simulink model "pgfm_ctrl_analysis"  (R2026b)
settings: Solver=ode23t  StopTime=param.sim.simlength  FixedStep=param.sim.tc  MaxStep=param.glb_time.tc  RelTol=1e-4
values from neighbouring files (symbols this model uses):
  param = add_template_extras(param, options)    [init_model.m]
undefined symbols (not defined in the file or in its folder): magnitude
libraries: fl_lib x99, nesl_utility x59, afe_uvw_ctrl x15, discrete_time_low_pass_filter x3, threephase_inductor_lib x3, dclink_for_two_levels x3, three_phase_pwm_modulator x3, ideal_bridges_lib x3, lithium_ion_battery x1, three_phase_voltage_with_frt_emulator_mfcn x1
(part 2 of 6)

== system pgfm_ctrl_analysis/grid/power meter iec mfunc ==
  Bus Selector : BusSelector  OutputSignals=Q1p,Q1n,P1n,P1p,U1n,U1p,i_act_1n,i_react_1n,i_act_1p,i_react_1p
  Constant : Constant  Value=param.glb_time.ts_afe
  Step : Step  Time=0.025  InitialValue=1  FinalValue=0  SampleTime=0
  To Workspace1 : ToWorkspace  VariableName=i_react_1n  SampleTime=param.glb_time.ts_afe
      settings: MaxDataPoints=param.glb_time.Ns_afe
  To Workspace2 : ToWorkspace  VariableName=i_react_1p  SampleTime=param.glb_time.ts_afe
      settings: MaxDataPoints=param.glb_time.Ns_afe
  To Workspace3 : ToWorkspace  VariableName=i_act_1n  SampleTime=param.glb_time.ts_afe
      settings: MaxDataPoints=param.glb_time.Ns_afe
  To Workspace4 : ToWorkspace  VariableName=i_act_1p  SampleTime=param.glb_time.ts_afe
      settings: MaxDataPoints=param.glb_time.Ns_afe
  To Workspace5 : ToWorkspace  VariableName=u1p  SampleTime=param.glb_time.ts_afe
      settings: MaxDataPoints=param.glb_time.Ns_afe
  To Workspace6 : ToWorkspace  VariableName=u1n  SampleTime=param.glb_time.ts_afe
      settings: MaxDataPoints=param.glb_time.Ns_afe
  Zero-Order Hold{,1..5} (6 alike) : ZeroOrderHold  SampleTime=param.glb_time.ts_afe
  three_phase_power_meter_iec : MATLAB Function  TreatAsAtomicUnit=on  SystemSampleTime=param.glb_time.ts_afe
  tag scope: P1n_global=global, P1p_global=global, Q1n_global=global, Q1p_global=global
  wires:
  Bus Selector/6 -> To Workspace5/1  "<U1p>"
  Bus Selector/8 -> To Workspace1/1  "<i_react_1n>"
  Bus Selector/10 -> To Workspace2/1  "<i_react_1p>"
  Bus Selector/5 -> To Workspace6/1  "<U1n>"
  Bus Selector/4 -> [P1p_global]  "<P1p>"
  Bus Selector/2 -> [Q1n_global]  "<Q1n>"
  Bus Selector/1 -> [Q1p_global]  "<Q1p>"
  Bus Selector/7 -> To Workspace3/1  "<i_act_1n>"
  Bus Selector/9 -> To Workspace4/1  "<i_act_1p>"
  Bus Selector/3 -> [P1n_global]  "<P1n>"
  three_phase_power_meter_iec/1(m) -> Bus Selector/1
  Zero-Order Hold/1 -> three_phase_power_meter_iec/1(phase)
  Zero-Order Hold2/1 -> three_phase_power_meter_iec/3(i_abc)
  [phase_grid_emulator] -> Zero-Order Hold/1
  Step/1 -> Zero-Order Hold5/1
  Zero-Order Hold3/1 -> three_phase_power_meter_iec/4(omega)
  Zero-Order Hold4/1 -> three_phase_power_meter_iec/5(ts)
  [ug_abc] -> Zero-Order Hold1/1
  Zero-Order Hold5/1 -> three_phase_power_meter_iec/6(enable_time)
  [ig_abc] -> Zero-Order Hold2/1
  [omega_grid_emulator] -> Zero-Order Hold3/1
  Constant/1 -> Zero-Order Hold4/1
  Zero-Order Hold1/1 -> three_phase_power_meter_iec/2(u_abc)

== system pgfm_ctrl_analysis/grid/threephase_vi_measures ==
  Bus Creator : BusCreator  Inputs=6
  Current Sensor : fl_lib/Electrical/Electrical Sensors/Current Sensor
  Current Sensor1 : fl_lib/Electrical/Electrical Sensors/Current Sensor
  Current Sensor2 : fl_lib/Electrical/Electrical Sensors/Current Sensor
  Electrical Reference1 : fl_lib/Electrical/Electrical Elements/Electrical Reference
  Selector : Selector  InputPortWidth=6  IndexOptions=Index vector (dialog)  Indices=[1 2 3]  OutputSizes=1  RuntimeRangeChecks=off
  Selector1 : Selector  InputPortWidth=6  IndexOptions=Index vector (dialog)  Indices=[4 5 6]  OutputSizes=1  RuntimeRangeChecks=off
  Voltage Sensor : fl_lib/Electrical/Electrical Sensors/Voltage Sensor
  Voltage Sensor1 : fl_lib/Electrical/Electrical Sensors/Voltage Sensor
  Voltage Sensor2 : fl_lib/Electrical/Electrical Sensors/Voltage Sensor
  ia_grid : nesl_utility/PS-Simulink Converter  PhysicalDomain=network_engine_domain  SubClassName=ps_output  LeftPortType=input  RightPortType=output  PseudoPeriodic=off  Frequencies=[]  VectorFormat=1-D array  Unit=A  AffineConversion=off
  ib_grid : nesl_utility/PS-Simulink Converter  PhysicalDomain=network_engine_domain  SubClassName=ps_output  LeftPortType=input  RightPortType=output  PseudoPeriodic=off  Frequencies=[]  VectorFormat=1-D array  Unit=A  AffineConversion=off
  ic_grid : nesl_utility/PS-Simulink Converter  PhysicalDomain=network_engine_domain  SubClassName=ps_output  LeftPortType=input  RightPortType=output  PseudoPeriodic=off  Frequencies=[]  VectorFormat=1-D array  Unit=A  AffineConversion=off
  ig_abc/ug_abc : Scope  NumInputPorts=2
      settings: SampleTime=param.glb_time.tc  ActiveDisplayYMinimum=-728.92703752654245  ActiveDisplayYMaximum=734.90808013997  DataLoggingVariableName=ScopeData2
  ua_grid : nesl_utility/PS-Simulink Converter  PhysicalDomain=network_engine_domain  SubClassName=ps_output  LeftPortType=input  RightPortType=output  PseudoPeriodic=off  Frequencies=[]  VectorFormat=1-D array  Unit=V  AffineConversion=off
  ub_grid : nesl_utility/PS-Simulink Converter  PhysicalDomain=network_engine_domain  SubClassName=ps_output  LeftPortType=input  RightPortType=output  PseudoPeriodic=off  Frequencies=[]  VectorFormat=1-D array  Unit=V  AffineConversion=off
  uc_grid : nesl_utility/PS-Simulink Converter  PhysicalDomain=network_engine_domain  SubClassName=ps_output  LeftPortType=input  RightPortType=output  PseudoPeriodic=off  Frequencies=[]  VectorFormat=1-D array  Unit=V  AffineConversion=off
  Ua : PMIOPort  Side=Left
  ua : PMIOPort  Port=2  Side=Right
  Ub : PMIOPort  Port=3  Side=Left
  ub : PMIOPort  Port=4  Side=Right
  Uc : PMIOPort  Port=5  Side=Left
  uc : PMIOPort  Port=6  Side=Right
  tag scope: ig_abc=global, ug_abc=global
  wires:
  Bus Creator/1 -> Selector1/1, Selector/1  "vi_data"
  Selector/1 -> [ug_abc]
  ib_grid/1 -> Bus Creator/5  "ib"
  ia_grid/1 -> Bus Creator/4  "ia"
  ic_grid/1 -> Bus Creator/6  "ic"
  ua_grid/1 -> Bus Creator/1  "ua"
  ub_grid/1 -> Bus Creator/2  "ub"
  uc_grid/1 -> Bus Creator/3  "uc"
  Selector1/1 -> [ig_abc]
  [ug_abc] -> ig_abc/ug_abc/2  "ug_abc(line)"
  [ig_abc] -> ig_abc/ug_abc/1  "ig_abc(line)"
  connections:
  Current Sensor1/LConn1 -- Ub/RConn1 -- Voltage Sensor1/LConn1
  Electrical Reference1/LConn1 -- Voltage Sensor/RConn2 -- Voltage Sensor2/RConn2 -- Voltage Sensor1/RConn2
  Voltage Sensor/RConn1 -- ua_grid/LConn1
  Current Sensor/RConn2 -- ua/RConn1
  Voltage Sensor1/RConn1 -- ub_grid/LConn1
  Voltage Sensor2/LConn1 -- Current Sensor2/LConn1 -- Uc/RConn1
  Current Sensor/LConn1 -- Ua/RConn1 -- Voltage Sensor/LConn1
  Current Sensor1/RConn2 -- ub/RConn1
  Voltage Sensor2/RConn1 -- uc_grid/LConn1
  ib_grid/LConn1 -- Current Sensor1/RConn1
  ia_grid/LConn1 -- Current Sensor/RConn1
  ic_grid/LConn1 -- Current Sensor2/RConn1
  Current Sensor2/RConn2 -- uc/RConn1

== system pgfm_ctrl_analysis/scopes/grid_afe_side ==
  Gain7 : Gain  Gain=param.afe.hw.ibez
  Gain8 : Gain  Gain=param.afe.hw.ubez
  Gain9 : Gain  Gain=param.afe.hw.ibez
  IEC_power_meter : Scope  NumInputPorts=4
      settings: ActiveDisplayYMinimum=-119219.77334314313  ActiveDisplayYMaximum=117736.49154199913  DataLoggingVariableName=ScopeData14
  i_line_abc/u_line_abc : Scope  NumInputPorts=2
      settings: SampleTime=param.glb_time.tc  ActiveDisplayYMinimum=-1413.9972740335056  ActiveDisplayYMaximum=1565.4749406115825  DataLoggingVariableName=ScopeData20
  idc/udc : Scope  NumInputPorts=2
      settings: SampleTime=param.glb_time.tc  ActiveDisplayYMinimum=-717.75084869622378  ActiveDisplayYMaximum=1484.0793366125047  DataLoggingVariableName=ScopeData23
  ig_abc/ug_abc _mod1 : Scope  NumInputPorts=2
      settings: SampleTime=param.glb_time.tc  ActiveDisplayYMinimum=-4.4957016262667837  ActiveDisplayYMaximum=4.3239423057982735  DataLoggingVariableName=ScopeData22
  is_abc/us_abc _mod1 : Scope  NumInputPorts=3
      settings: SampleTime=param.glb_time.tc  ActiveDisplayYMinimum=-1452.0325690620477  ActiveDisplayYMaximum=1524.1423010817562  DataLoggingVariableName=ScopeData21
  udc voltages : Scope  NumInputPorts=2
      settings: SampleTime=param.glb_time.tc  ActiveDisplayYMinimum=-0.15419783204284679  ActiveDisplayYMaximum=1.3782838496471517  DataLoggingVariableName=ScopeData24
  wires:
  [udc_mod1] -> idc/udc/2  "udc_dclink_mod1"
  [ug_abc_pu_mod1] -> ig_abc/ug_abc _mod1/2  "ug_abc_mod1"
  Gain8/1 -> is_abc/us_abc _mod1/2  "vs_abc_mod1"
  [ic_dclink_mod1] -> idc/udc/1  "ic_dclink_mod1"
  [is_abc_pu_mod1] -> Gain7/1
  [Q1p_global] -> IEC_power_meter/2  "Q1p_global"
  [all_voltages_about_dclink] -> udc voltages/2  "all_voltages_about_dclink"
  Gain7/1 -> is_abc/us_abc _mod1/1  "is_abc_mod1"
  [iz_afe_pu_mod1] -> Gain9/1
  [i_abc_line] -> i_line_abc/u_line_abc/1  "i_abc_line"
  [u_abc_line] -> i_line_abc/u_line_abc/2  "u_abc_line"
  [P1n_global] -> IEC_power_meter/4  "P1n_global"
  [ig_abc_pu_mod1] -> ig_abc/ug_abc _mod1/1  "ig_abc_mod1"
  [vs_abc_pu_mod1] -> Gain8/1
  [vdc_pu_afe_mod1] -> udc voltages/1  "udc"
  Gain9/1 -> is_abc/us_abc _mod1/3  "iz_afe_mod1"
  [Q1n_global] -> IEC_power_meter/1  "Q1n_global"
  [P1p_global] -> IEC_power_meter/3  "P1p_global"

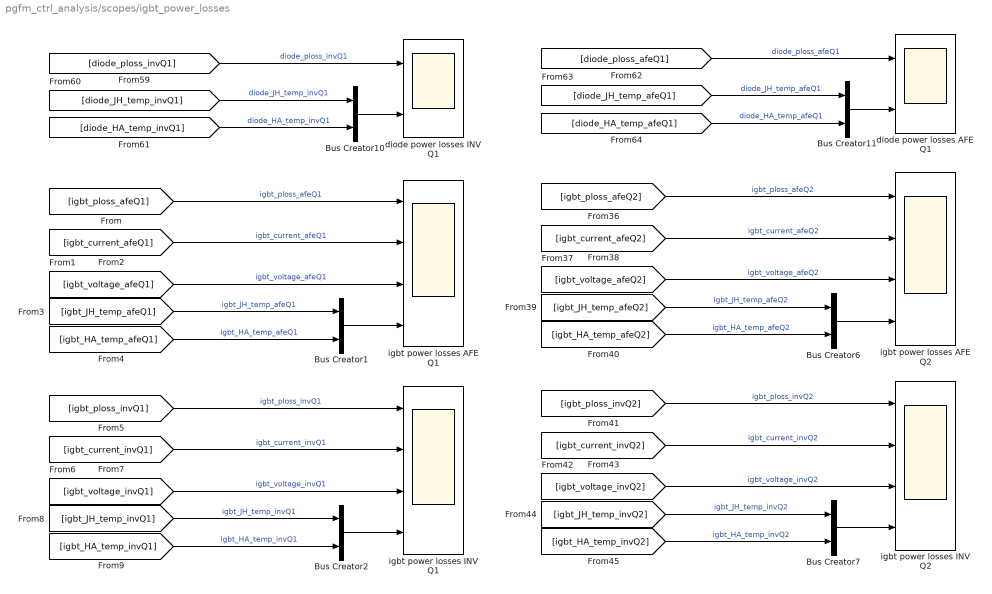
== system pgfm_ctrl_analysis/scopes/igbt_power_losses ==
  Bus Creator{1..2,6..7,10..11} (6 alike) : BusCreator  Inputs=2
  diode power losses AFE Q1 : Scope  NumInputPorts=2
      settings: SampleTime=param.glb_time.tc  ActiveDisplayYMinimum=-0.87039317174009745  ActiveDisplayYMaximum=7.8312553964690395  DataLoggingVariableName=ScopeData32
  diode power losses INV Q1 : Scope  NumInputPorts=2
      settings: SampleTime=param.glb_time.tc  ActiveDisplayYMinimum=-1  ActiveDisplayYMaximum=1  DataLoggingVariableName=ScopeData31
  igbt power losses AFE Q1 : Scope  NumInputPorts=4
      settings: SampleTime=param.glb_time.tc  ActiveDisplayYMinimum=-49.038943467813  ActiveDisplayYMaximum=441.3504912103171  DataLoggingVariableName=ScopeData15
  igbt power losses AFE Q2 : Scope  NumInputPorts=4
      settings: SampleTime=param.glb_time.tc  ActiveDisplayYMinimum=-40.410135398015626  ActiveDisplayYMaximum=363.69121858214072  DataLoggingVariableName=ScopeData26
  igbt power losses INV Q1 : Scope  NumInputPorts=4
      settings: SampleTime=param.glb_time.tc  ActiveDisplayYMinimum=-36.37444736851036  ActiveDisplayYMaximum=327.37002631659328  DataLoggingVariableName=ScopeData16
  igbt power losses INV Q2 : Scope  NumInputPorts=4
      settings: SampleTime=param.glb_time.tc  ActiveDisplayYMinimum=-6409.6577502266955  ActiveDisplayYMaximum=762.94403267363941  DataLoggingVariableName=ScopeData27
  wires:
  [igbt_ploss_afeQ1] -> igbt power losses AFE Q1/1  "igbt_ploss_afeQ1"
  [igbt_JH_temp_invQ1] -> Bus Creator2/1  "igbt_JH_temp_invQ1"
  [diode_JH_temp_invQ1] -> Bus Creator10/1  "diode_JH_temp_invQ1"
  [igbt_HA_temp_invQ2] -> Bus Creator7/2  "igbt_HA_temp_invQ2"
  [igbt_current_afeQ2] -> igbt power losses AFE Q2/2  "igbt_current_afeQ2"
  [igbt_ploss_afeQ2] -> igbt power losses AFE Q2/1  "igbt_ploss_afeQ2"
  [igbt_current_invQ1] -> igbt power losses INV Q1/2  "igbt_current_invQ1"
  [igbt_JH_temp_afeQ1] -> Bus Creator1/1  "igbt_JH_temp_afeQ1"
  [igbt_current_invQ2] -> igbt power losses INV Q2/2  "igbt_current_invQ2"
  [diode_JH_temp_afeQ1] -> Bus Creator11/1  "diode_JH_temp_afeQ1"
  [igbt_HA_temp_invQ1] -> Bus Creator2/2  "igbt_HA_temp_invQ1"
  [igbt_JH_temp_afeQ2] -> Bus Creator6/1  "igbt_JH_temp_afeQ2"
  Bus Creator11/1 -> diode power losses AFE Q1/2
  [diode_ploss_invQ1] -> diode power losses INV Q1/1  "diode_ploss_invQ1"
  [igbt_ploss_invQ1] -> igbt power losses INV Q1/1  "igbt_ploss_invQ1"
  [igbt_HA_temp_afeQ2] -> Bus Creator6/2  "igbt_HA_temp_afeQ2"
  Bus Creator7/1 -> igbt power losses INV Q2/4
  [igbt_voltage_invQ2] -> igbt power losses INV Q2/3  "igbt_voltage_invQ2"
  Bus Creator10/1 -> diode power losses INV Q1/2
  [igbt_JH_temp_invQ2] -> Bus Creator7/1  "igbt_JH_temp_invQ2"
  [diode_HA_temp_afeQ1] -> Bus Creator11/2  "diode_HA_temp_afeQ1"
  Bus Creator1/1 -> igbt power losses AFE Q1/4
  Bus Creator6/1 -> igbt power losses AFE Q2/4
  [igbt_voltage_afeQ1] -> igbt power losses AFE Q1/3  "igbt_voltage_afeQ1"
  [igbt_current_afeQ1] -> igbt power losses AFE Q1/2  "igbt_current_afeQ1"
  [igbt_HA_temp_afeQ1] -> Bus Creator1/2  "igbt_HA_temp_afeQ1"
  [diode_ploss_afeQ1] -> diode power losses AFE Q1/1  "diode_ploss_afeQ1"
  Bus Creator2/1 -> igbt power losses INV Q1/4
  [diode_HA_temp_invQ1] -> Bus Creator10/2  "diode_HA_temp_invQ1"
  [igbt_voltage_invQ1] -> igbt power losses INV Q1/3  "igbt_voltage_invQ1"
  [igbt_ploss_invQ2] -> igbt power losses INV Q2/1  "igbt_ploss_invQ2"
  [igbt_voltage_afeQ2] -> igbt power losses AFE Q2/3  "igbt_voltage_afeQ2"

== system pgfm_ctrl_analysis/scopes/mosfet_power_losses ==
  Bus Creator8 : BusCreator  Inputs=2
  Bus Creator9 : BusCreator  Inputs=2
  mosfet power losses INV Q1 : Scope  NumInputPorts=4
      settings: SampleTime=param.glb_time.tc  ActiveDisplayYMinimum=-52.647210306071649  ActiveDisplayYMaximum=473.81757031333393  DataLoggingVariableName=ScopeData28
  mosfet power losses INV Q2 : Scope  NumInputPorts=4
      settings: SampleTime=param.glb_time.tc  ActiveDisplayYMinimum=-60.051099059926763  ActiveDisplayYMaximum=540.45256909803  DataLoggingVariableName=ScopeData29
  wires:
  [mosfet_current_invQ2] -> mosfet power losses INV Q2/3  "mosfet_current_invQ2"
  [mosfet_voltage_invQ1] -> mosfet power losses INV Q1/2  "mosfet_voltage_invQ1"
  [mosfet_HA_temp_invQ2] -> Bus Creator9/2  "mosfet_HA_temp_invQ2"
  [mosfet_JH_temp_invQ2] -> Bus Creator9/1  "mosfet_JH_temp_invQ2"
  [mosfet_ploss_invQ1] -> mosfet power losses INV Q1/1  "mosfet_ploss_invQ1"
  [mosfet_HA_temp_invQ1] -> Bus Creator8/2  "mosfet_HA_temp_invQ1"
  [mosfet_current_invQ1] -> mosfet power losses INV Q1/3  "mosfet_current_invQ1"
  Bus Creator8/1 -> mosfet power losses INV Q1/4
  [mosfet_voltage_invQ2] -> mosfet power losses INV Q2/2  "mosfet_voltage_invQ2"
  [mosfet_ploss_invQ2] -> mosfet power losses INV Q2/1  "mosfet_ploss_invQ2"
  Bus Creator9/1 -> mosfet power losses INV Q2/4
  [mosfet_JH_temp_invQ1] -> Bus Creator8/1  "mosfet_JH_temp_invQ1"

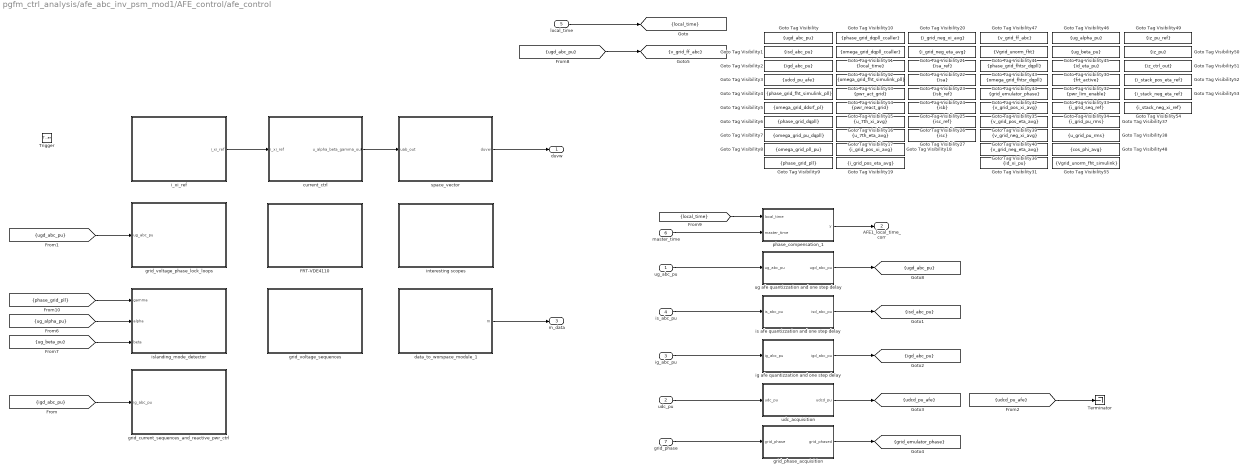
== system pgfm_ctrl_analysis/afe_abc_inv_psm_mod1/AFE_control/afe_control ==
  ug_abc_pu : Inport
  udc_pu : Inport  Port=2
  ig_abc_pu : Inport  Port=3
  is_abc_pu : Inport  Port=4
  local_time : Inport  Port=5
  master_time : Inport  Port=6
  grid_phase : Inport  Port=7
  Trigger : TriggerPort  VariantControl=(inherit)  PortDimensions=1
  FRT-VDE4110 : Subsystem
  Goto Tag Visibility : GotoTagVisibility  GotoTag=ugd_abc_pu
  Goto Tag Visibility1 : GotoTagVisibility  GotoTag=isd_abc_pu
  Goto Tag Visibility10 : GotoTagVisibility  GotoTag=phase_grid_dqpll_ccaller
  Goto Tag Visibility11 : GotoTagVisibility  GotoTag=omega_grid_dqpll_ccaller
  Goto Tag Visibility12 : GotoTagVisibility  GotoTag=local_time
  Goto Tag Visibility13 : GotoTagVisibility  GotoTag=omega_grid_fht_simulink_pll
  Goto Tag Visibility14 : GotoTagVisibility  GotoTag=pwr_act_grid
  Goto Tag Visibility15 : GotoTagVisibility  GotoTag=pwr_react_grid
  Goto Tag Visibility16 : GotoTagVisibility  GotoTag=u_7th_xi_avg
  Goto Tag Visibility17 : GotoTagVisibility  GotoTag=u_7th_eta_avg
  Goto Tag Visibility18 : GotoTagVisibility  GotoTag=i_grid_pos_xi_avg
  Goto Tag Visibility19 : GotoTagVisibility  GotoTag=i_grid_pos_eta_avg
  Goto Tag Visibility2 : GotoTagVisibility  GotoTag=igd_abc_pu
  Goto Tag Visibility20 : GotoTagVisibility  GotoTag=i_grid_neg_xi_avg
  Goto Tag Visibility21 : GotoTagVisibility  GotoTag=i_grid_neg_eta_avg
  Goto Tag Visibility22 : GotoTagVisibility  GotoTag=isa_ref
  Goto Tag Visibility23 : GotoTagVisibility  GotoTag=isa
  Goto Tag Visibility24 : GotoTagVisibility  GotoTag=isb_ref
  Goto Tag Visibility25 : GotoTagVisibility  GotoTag=isb
  Goto Tag Visibility26 : GotoTagVisibility  GotoTag=isc_ref
  Goto Tag Visibility27 : GotoTagVisibility  GotoTag=isc
  Goto Tag Visibility3 : GotoTagVisibility  GotoTag=udcd_pu_afe
  Goto Tag Visibility30 : GotoTagVisibility  GotoTag=id_eta_pu
  Goto Tag Visibility31 : GotoTagVisibility  GotoTag=id_xi_pu
  Goto Tag Visibility32 : GotoTagVisibility  GotoTag=frt_active
  Goto Tag Visibility33 : GotoTagVisibility  GotoTag=pwr_lim_enable
  Goto Tag Visibility34 : GotoTagVisibility  GotoTag=i_grid_seq_ref
  Goto Tag Visibility35 : GotoTagVisibility  GotoTag=v_grid_pos_xi_avg
  Goto Tag Visibility36 : GotoTagVisibility  GotoTag=v_grid_neg_eta_avg
  Goto Tag Visibility37 : GotoTagVisibility  GotoTag=i_grid_pu_rms
  Goto Tag Visibility38 : GotoTagVisibility  GotoTag=u_grid_pu_rms
  Goto Tag Visibility39 : GotoTagVisibility  GotoTag=v_grid_pos_eta_avg
  Goto Tag Visibility4 : GotoTagVisibility  GotoTag=phase_grid_fht_simulink_pll
  Goto Tag Visibility40 : GotoTagVisibility  GotoTag=v_grid_neg_xi_avg
  Goto Tag Visibility41 : GotoTagVisibility  GotoTag=Vgrid_unorm_fht
  Goto Tag Visibility42 : GotoTagVisibility  GotoTag=grid_emulator_phase
  Goto Tag Visibility43 : GotoTagVisibility  GotoTag=phase_grid_fhtsr_dqpll
  Goto Tag Visibility44 : GotoTagVisibility  GotoTag=omega_grid_fhtsr_dqpll
  Goto Tag Visibility45 : GotoTagVisibility  GotoTag=ug_beta_pu
  Goto Tag Visibility46 : GotoTagVisibility  GotoTag=ug_alpha_pu
  Goto Tag Visibility47 : GotoTagVisibility  GotoTag=v_grid_ff_abc
  Goto Tag Visibility48 : GotoTagVisibility  GotoTag=cos_phi_avg
  Goto Tag Visibility49 : GotoTagVisibility  GotoTag=iz_pu_ref
  Goto Tag Visibility5 : GotoTagVisibility  GotoTag=omega_grid_ddsrf_pl
  Goto Tag Visibility50 : GotoTagVisibility  GotoTag=iz_pu
  Goto Tag Visibility51 : GotoTagVisibility  GotoTag=iz_ctrl_out
  Goto Tag Visibility52 : GotoTagVisibility  GotoTag=i_stack_pos_eta_ref
  Goto Tag Visibility53 : GotoTagVisibility  GotoTag=i_stack_neg_eta_ref
  Goto Tag Visibility54 : GotoTagVisibility  GotoTag=i_stack_neg_xi_ref
  Goto Tag Visibility55 : GotoTagVisibility  GotoTag=Vgrid_unorm_fht_simulink
  Goto Tag Visibility6 : GotoTagVisibility  GotoTag=phase_grid_dqpll
  Goto Tag Visibility7 : GotoTagVisibility  GotoTag=omega_grid_pu_dqpll
  Goto Tag Visibility8 : GotoTagVisibility  GotoTag=omega_grid_pll_pu
  Goto Tag Visibility9 : GotoTagVisibility  GotoTag=phase_grid_pll
  Terminator : Terminator
  current_ctrl : Subsystem
  data_to_worspace_module_1 : Subsystem
  grid_current_sequences_and_reactive_pwr_ctrl : Subsystem
  grid_phase_acquisition : Subsystem
  grid_voltage_phase_lock_loops : Subsystem
  grid_voltage_sequences : Subsystem
  i_xi_ref : Subsystem
  ig afe quantizzation and one step delay : Subsystem
  interesting scopes : Subsystem
  is afe quantizzation and one step delay : Subsystem
  islanding_mode_detector : Subsystem
  phase_compensation_1 : Subsystem
  space_vector : Subsystem
  udc_acquisition : Subsystem
  ug afe quantizzation and one step delay : Subsystem
  duvw : Outport
  AFE1_local_time_corr : Outport  Port=2
  m_data : Outport  Port=3
  tag scope: grid_emulator_phase=scoped, igd_abc_pu=scoped, isd_abc_pu=scoped, local_time=scoped, udcd_pu_afe=scoped, ugd_abc_pu=scoped, v_grid_ff_abc=scoped
  wires:
  ug_abc_pu/1 -> ug afe quantizzation and one step delay/1(ug_abc_pu)
  space_vector/1(duvw) -> duvw/1
  is_abc_pu/1 -> is afe quantizzation and one step delay/1(is_abc_pu)
  ig_abc_pu/1 -> ig afe quantizzation and one step delay/1(ig_abc_pu)
  [ugd_abc_pu] -> grid_voltage_phase_lock_loops/1(ug_abc_pu)
  [igd_abc_pu] -> grid_current_sequences_and_reactive_pwr_ctrl/1(ig_abc_pu)
  udc_pu/1 -> udc_acquisition/1(udc_pu)
  udc_acquisition/1(udcd_pu) -> [udcd_pu_afe]
  [phase_grid_pll] -> islanding_mode_detector/1(gamma)
  [ug_alpha_pu] -> islanding_mode_detector/2(alpha)
  ug afe quantizzation and one step delay/1(ugd_abc_pu) -> [ugd_abc_pu]
  is afe quantizzation and one step delay/1(isd_abc_pu) -> [isd_abc_pu]
  ig afe quantizzation and one step delay/1(igd_abc_pu) -> [igd_abc_pu]
  [ug_beta_pu] -> islanding_mode_detector/3(beta)
  local_time/1 -> [local_time]
  master_time/1 -> phase_compensation_1/2(master_time)
  phase_compensation_1/1(y) -> AFE1_local_time_corr/1
  [local_time] -> phase_compensation_1/1(local_time)
  grid_phase/1 -> grid_phase_acquisition/1(grid_phase)
  grid_phase_acquisition/1(grid_phased) -> [grid_emulator_phase]
  [ugd_abc_pu] -> [v_grid_ff_abc]
  data_to_worspace_module_1/1(m) -> m_data/1
  [udcd_pu_afe] -> Terminator/1
  current_ctrl/1(u_alpha_beta_gamma_out) -> space_vector/1(uab_out)
  i_xi_ref/1(i_xi_ref) -> current_ctrl/1(i_xi_ref)

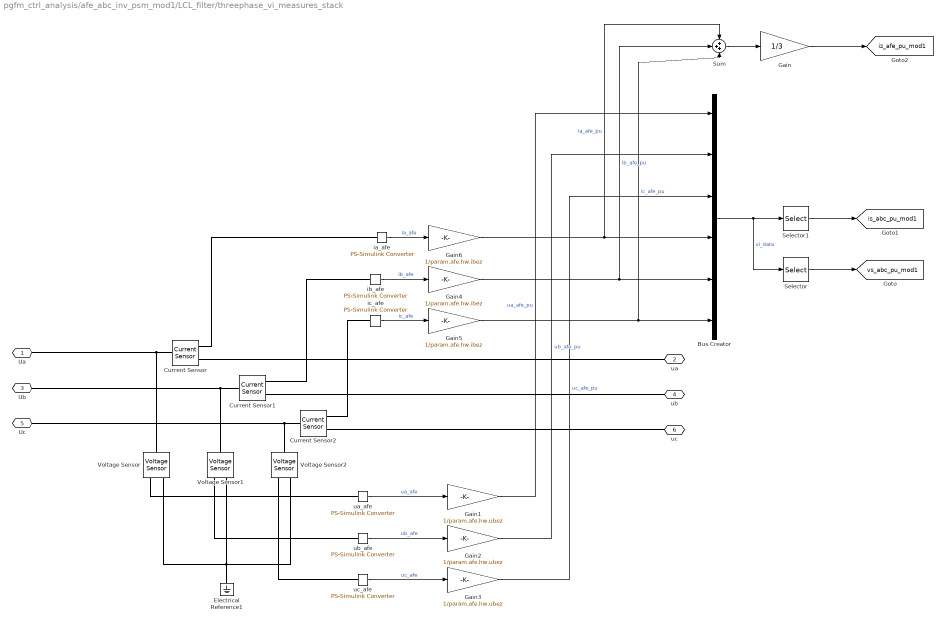
== system pgfm_ctrl_analysis/afe_abc_inv_psm_mod1/LCL_filter/threephase_vi_measures_stack ==
  Bus Creator : BusCreator  Inputs=6
  Current Sensor : fl_lib/Electrical/Electrical Sensors/Current Sensor
  Current Sensor1 : fl_lib/Electrical/Electrical Sensors/Current Sensor
  Current Sensor2 : fl_lib/Electrical/Electrical Sensors/Current Sensor
  Electrical Reference1 : fl_lib/Electrical/Electrical Elements/Electrical Reference
  Gain : Gain  Gain=1/3
  Gain1 : Gain  Gain=1/param.afe.hw.ubez
  Gain2 : Gain  Gain=1/param.afe.hw.ubez
  Gain3 : Gain  Gain=1/param.afe.hw.ubez
  Gain4 : Gain  Gain=1/param.afe.hw.ibez
  Gain5 : Gain  Gain=1/param.afe.hw.ibez
  Gain6 : Gain  Gain=1/param.afe.hw.ibez
  Selector : Selector  InputPortWidth=6  IndexOptions=Index vector (dialog)  Indices=[1 2 3]  OutputSizes=1  RuntimeRangeChecks=off
  Selector1 : Selector  InputPortWidth=6  IndexOptions=Index vector (dialog)  Indices=[4 5 6]  OutputSizes=1  RuntimeRangeChecks=off
  Sum : Sum  Inputs=+++
  Voltage Sensor : fl_lib/Electrical/Electrical Sensors/Voltage Sensor
  Voltage Sensor1 : fl_lib/Electrical/Electrical Sensors/Voltage Sensor
  Voltage Sensor2 : fl_lib/Electrical/Electrical Sensors/Voltage Sensor
  ia_afe : nesl_utility/PS-Simulink Converter  PhysicalDomain=network_engine_domain  SubClassName=ps_output  LeftPortType=input  RightPortType=output  PseudoPeriodic=off  Frequencies=[]  VectorFormat=1-D array  Unit=A  AffineConversion=off
  ib_afe : nesl_utility/PS-Simulink Converter  PhysicalDomain=network_engine_domain  SubClassName=ps_output  LeftPortType=input  RightPortType=output  PseudoPeriodic=off  Frequencies=[]  VectorFormat=1-D array  Unit=A  AffineConversion=off
  ic_afe : nesl_utility/PS-Simulink Converter  PhysicalDomain=network_engine_domain  SubClassName=ps_output  LeftPortType=input  RightPortType=output  PseudoPeriodic=off  Frequencies=[]  VectorFormat=1-D array  Unit=A  AffineConversion=off
  ua_afe : nesl_utility/PS-Simulink Converter  PhysicalDomain=network_engine_domain  SubClassName=ps_output  LeftPortType=input  RightPortType=output  PseudoPeriodic=off  Frequencies=[]  VectorFormat=1-D array  Unit=V  AffineConversion=off
  ub_afe : nesl_utility/PS-Simulink Converter  PhysicalDomain=network_engine_domain  SubClassName=ps_output  LeftPortType=input  RightPortType=output  PseudoPeriodic=off  Frequencies=[]  VectorFormat=1-D array  Unit=V  AffineConversion=off
  uc_afe : nesl_utility/PS-Simulink Converter  PhysicalDomain=network_engine_domain  SubClassName=ps_output  LeftPortType=input  RightPortType=output  PseudoPeriodic=off  Frequencies=[]  VectorFormat=1-D array  Unit=V  AffineConversion=off
  Ua : PMIOPort  Side=Left
  ua : PMIOPort  Port=2  Side=Right
  Ub : PMIOPort  Port=3  Side=Left
  ub : PMIOPort  Port=4  Side=Right
  Uc : PMIOPort  Port=5  Side=Left
  uc : PMIOPort  Port=6  Side=Right
  tag scope: is_abc_pu_mod1=global, iz_afe_pu_mod1=global, vs_abc_pu_mod1=global
  wires:
  Bus Creator/1 -> Selector/1, Selector1/1  "vi_data"
  Selector/1 -> [vs_abc_pu_mod1]
  ib_afe/1 -> Gain4/1  "ib_afe"
  ia_afe/1 -> Gain6/1  "ia_afe"
  ic_afe/1 -> Gain5/1  "ic_afe"
  ua_afe/1 -> Gain1/1  "ua_afe"
  ub_afe/1 -> Gain2/1  "ub_afe"
  uc_afe/1 -> Gain3/1  "uc_afe"
  Selector1/1 -> [is_abc_pu_mod1]
  Sum/1 -> Gain/1
  Gain/1 -> [iz_afe_pu_mod1]
  Gain1/1 -> Bus Creator/1  "ua_afe_pu"
  Gain2/1 -> Bus Creator/2  "ub_afe_pu"
  Gain3/1 -> Bus Creator/3  "uc_afe_pu"
  Gain6/1 -> Sum/1, Bus Creator/4  "ia_afe_pu"
  Gain4/1 -> Sum/2, Bus Creator/5  "ib_afe_pu"
  Gain5/1 -> Bus Creator/6, Sum/3  "ic_afe_pu"
  connections:
  Current Sensor1/LConn1 -- Ub/RConn1 -- Voltage Sensor1/LConn1
  Electrical Reference1/LConn1 -- Voltage Sensor/RConn2 -- Voltage Sensor2/RConn2 -- Voltage Sensor1/RConn2
  Voltage Sensor/RConn1 -- ua_afe/LConn1
  Current Sensor/RConn2 -- ua/RConn1
  Voltage Sensor1/RConn1 -- ub_afe/LConn1
  Voltage Sensor2/LConn1 -- Uc/RConn1 -- Current Sensor2/LConn1
  Current Sensor/LConn1 -- Ua/RConn1 -- Voltage Sensor/LConn1
  Current Sensor1/RConn2 -- ub/RConn1
  Voltage Sensor2/RConn1 -- uc_afe/LConn1
  ib_afe/LConn1 -- Current Sensor1/RConn1
  ia_afe/LConn1 -- Current Sensor/RConn1
  ic_afe/LConn1 -- Current Sensor2/RConn1
  Current Sensor2/RConn2 -- uc/RConn1

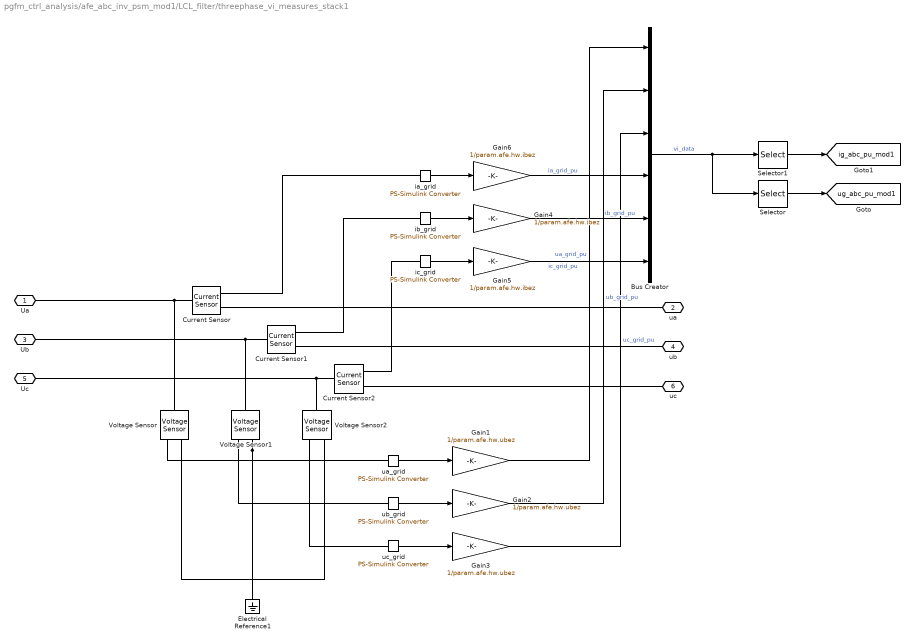
== system pgfm_ctrl_analysis/afe_abc_inv_psm_mod1/LCL_filter/threephase_vi_measures_stack1 ==
  Bus Creator : BusCreator  Inputs=6
  Current Sensor : fl_lib/Electrical/Electrical Sensors/Current Sensor
  Current Sensor1 : fl_lib/Electrical/Electrical Sensors/Current Sensor
  Current Sensor2 : fl_lib/Electrical/Electrical Sensors/Current Sensor
  Electrical Reference1 : fl_lib/Electrical/Electrical Elements/Electrical Reference
  Gain1 : Gain  Gain=1/param.afe.hw.ubez
  Gain2 : Gain  Gain=1/param.afe.hw.ubez
  Gain3 : Gain  Gain=1/param.afe.hw.ubez
  Gain4 : Gain  Gain=1/param.afe.hw.ibez
  Gain5 : Gain  Gain=1/param.afe.hw.ibez
  Gain6 : Gain  Gain=1/param.afe.hw.ibez
  Selector : Selector  InputPortWidth=6  IndexOptions=Index vector (dialog)  Indices=[1 2 3]  OutputSizes=1  RuntimeRangeChecks=off
  Selector1 : Selector  InputPortWidth=6  IndexOptions=Index vector (dialog)  Indices=[4 5 6]  OutputSizes=1  RuntimeRangeChecks=off
  Voltage Sensor : fl_lib/Electrical/Electrical Sensors/Voltage Sensor
  Voltage Sensor1 : fl_lib/Electrical/Electrical Sensors/Voltage Sensor
  Voltage Sensor2 : fl_lib/Electrical/Electrical Sensors/Voltage Sensor
  ia_grid : nesl_utility/PS-Simulink Converter  PhysicalDomain=network_engine_domain  SubClassName=ps_output  LeftPortType=input  RightPortType=output  PseudoPeriodic=off  Frequencies=[]  VectorFormat=1-D array  Unit=A  AffineConversion=off
  ib_grid : nesl_utility/PS-Simulink Converter  PhysicalDomain=network_engine_domain  SubClassName=ps_output  LeftPortType=input  RightPortType=output  PseudoPeriodic=off  Frequencies=[]  VectorFormat=1-D array  Unit=A  AffineConversion=off
  ic_grid : nesl_utility/PS-Simulink Converter  PhysicalDomain=network_engine_domain  SubClassName=ps_output  LeftPortType=input  RightPortType=output  PseudoPeriodic=off  Frequencies=[]  VectorFormat=1-D array  Unit=A  AffineConversion=off
  ua_grid : nesl_utility/PS-Simulink Converter  PhysicalDomain=network_engine_domain  SubClassName=ps_output  LeftPortType=input  RightPortType=output  PseudoPeriodic=off  Frequencies=[]  VectorFormat=1-D array  Unit=V  AffineConversion=off
  ub_grid : nesl_utility/PS-Simulink Converter  PhysicalDomain=network_engine_domain  SubClassName=ps_output  LeftPortType=input  RightPortType=output  PseudoPeriodic=off  Frequencies=[]  VectorFormat=1-D array  Unit=V  AffineConversion=off
  uc_grid : nesl_utility/PS-Simulink Converter  PhysicalDomain=network_engine_domain  SubClassName=ps_output  LeftPortType=input  RightPortType=output  PseudoPeriodic=off  Frequencies=[]  VectorFormat=1-D array  Unit=V  AffineConversion=off
  Ua : PMIOPort  Side=Left
  ua : PMIOPort  Port=2  Side=Right
  Ub : PMIOPort  Port=3  Side=Left
  ub : PMIOPort  Port=4  Side=Right
  Uc : PMIOPort  Port=5  Side=Left
  uc : PMIOPort  Port=6  Side=Right
  tag scope: ig_abc_pu_mod1=global, ug_abc_pu_mod1=global
  wires:
  Selector1/1 -> [ig_abc_pu_mod1]
  uc_grid/1 -> Gain3/1
  ub_grid/1 -> Gain2/1
  ua_grid/1 -> Gain1/1
  ic_grid/1 -> Gain5/1
  ia_grid/1 -> Gain6/1
  ib_grid/1 -> Gain4/1
  Selector/1 -> [ug_abc_pu_mod1]
  Bus Creator/1 -> Selector1/1, Selector/1  "vi_data"
  Gain1/1 -> Bus Creator/1  "ua_grid_pu"
  Gain2/1 -> Bus Creator/2  "ub_grid_pu"
  Gain3/1 -> Bus Creator/3  "uc_grid_pu"
  Gain6/1 -> Bus Creator/4  "ia_grid_pu"
  Gain4/1 -> Bus Creator/5  "ib_grid_pu"
  Gain5/1 -> Bus Creator/6  "ic_grid_pu"
  connections:
  Current Sensor2/RConn2 -- uc/RConn1
  ic_grid/LConn1 -- Current Sensor2/RConn1
  ia_grid/LConn1 -- Current Sensor/RConn1
  ib_grid/LConn1 -- Current Sensor1/RConn1
  Voltage Sensor2/RConn1 -- uc_grid/LConn1
  Current Sensor1/RConn2 -- ub/RConn1
  Voltage Sensor/LConn1 -- Current Sensor/LConn1 -- Ua/RConn1
  Current Sensor2/LConn1 -- Voltage Sensor2/LConn1 -- Uc/RConn1
  Voltage Sensor1/RConn1 -- ub_grid/LConn1
  Current Sensor/RConn2 -- ua/RConn1
  Voltage Sensor/RConn1 -- ua_grid/LConn1
  Voltage Sensor1/RConn2 -- Voltage Sensor2/RConn2 -- Voltage Sensor/RConn2 -- Electrical Reference1/LConn1
  Voltage Sensor1/LConn1 -- Current Sensor1/LConn1 -- Ub/RConn1

== system pgfm_ctrl_analysis/afe_abc_inv_psm_mod1/afe/sv_pwm ==
  duties_uvw : Inport
  Bus Selector2 : BusSelector  OutputSignals=du(k),dv(k),dw(k)
  Constant1 : Constant  Value=param.afe.behav.pwm_phase_shift_mod1
  modulator1 : Subsystem
  td2tc_1 : TransferFcn  Denominator=[param.glb_time.tc 1]
  td2tc_2 : TransferFcn  Denominator=[param.glb_time.tc 1]
  td2tc_3 : TransferFcn  Denominator=[param.glb_time.tc 1]
  gate_cmds : Outport
  wires:
  modulator1/1(gate_cmds) -> gate_cmds/1
  Constant1/1 -> modulator1/4(phase)
  Bus Selector2/1 -> td2tc_1/1  "<du(k)>"
  Bus Selector2/2 -> td2tc_2/1  "<dv(k)>"
  Bus Selector2/3 -> td2tc_3/1  "<dw(k)>"
  duties_uvw/1 -> Bus Selector2/1
  td2tc_1/1 -> modulator1/1(u)  "du(t)"
  td2tc_3/1 -> modulator1/3(w)  "dw(t)"
  td2tc_2/1 -> modulator1/2(v)  "dv(t)"

== system pgfm_ctrl_analysis/afe_abc_inv_psm_mod1/afe/three_phase_inverter_ideal_switch_based_model ==
  gate_commands : Inport
  PS Terminator : fl_lib/Physical Signals/Sinks/PS Terminator
  PS Terminator1 : fl_lib/Physical Signals/Sinks/PS Terminator
  Simulink-PS Converter : nesl_utility/Simulink-PS Converter  PhysicalDomain=network_engine_domain  SubClassName=ps_input  LeftPortType=input  RightPortType=output  PseudoPeriodic=off  Frequencies=[]  NoiseDistribution=none  NoiseParameters=[]  Unit=V  AffineConversion=off  FilteringAndDerivatives=provide  SimscapeFilterOrder=1  InputFilterTimeConstant=0.001  UdotUserProvided=0
  Three-Phase Bridge (ideal) : ideal_bridges_lib/Three-Phase Bridge (ideal)  Vth=2.5 V  Ron=1e-3 Ohm  Goff=1e-6 1/Ohm  cap_dc=ideal_bridges.onoff.on  Cdc=2e-3 F  Vdc0=0 V  ind_ac=ideal_bridges.onoff.on  L=1e-3 H  RL=10e-3 Ohm  vdc_specify=off  vdc_priority=None  vdc=0 V  vdc_nominal_specify=off  vdc_nominal_value=1  vdc_nominal_unit=V  ic_specify=off  ic_priority=None  ic=0 A  ic_nominal_specify=off  ic_nominal_value=1  ic_nominal_unit=A  vm_a_specify=off  vm_a_priority=None  vm_a=0 V  vm_a_nominal_specify=off  vm_a_nominal_value=1  vm_a_nominal_unit=V  vm_b_specify=off  vm_b_priority=None  vm_b=0 V  vm_b_nominal_specify=off  vm_b_nominal_value=1  vm_b_nominal_unit=V  vm_c_specify=off  vm_c_priority=None  vm_c=0 V  vm_c_nominal_specify=off  vm_c_nominal_value=1  vm_c_nominal_unit=V  i_ah_specify=off  i_ah_priority=None  i_ah=0 A  i_ah_nominal_specify=off  i_ah_nominal_value=1  i_ah_nominal_unit=A  i_al_specify=off  i_al_priority=None  i_al=0 A  i_al_nominal_specify=off  i_al_nominal_value=1  i_al_nominal_unit=A  i_bh_specify=off  i_bh_priority=None  i_bh=0 A  i_bh_nominal_specify=off  i_bh_nominal_value=1  i_bh_nominal_unit=A  i_bl_specify=off  i_bl_priority=None  i_bl=0 A  i_bl_nominal_specify=off  i_bl_nominal_value=1  i_bl_nominal_unit=A  i_ch_specify=off  i_ch_priority=None  i_ch=0 A  i_ch_nominal_specify=off  i_ch_nominal_value=1  i_ch_nominal_unit=A  i_cl_specify=off  i_cl_priority=None  i_cl=0 A  i_cl_nominal_specify=off  i_cl_nominal_value=1  i_cl_nominal_unit=A  i_a_specify=off  i_a_priority=None  i_a=0 A  i_a_nominal_specify=off  i_a_nominal_value=1  i_a_nominal_unit=A  i_b_specify=off  i_b_priority=None  i_b=0 A  i_b_nominal_specify=off  i_b_nominal_value=1  i_b_nominal_unit=A  i_c_specify=off  i_c_priority=None  i_c=0 A  i_c_nominal_specify=off  i_c_nominal_value=1  i_c_nominal_unit=A
  udc(+) : PMIOPort  Side=Left
  u : PMIOPort  Port=2  Side=Right
  v : PMIOPort  Port=3  Side=Right
  udc(-) : PMIOPort  Port=4  Side=Left
  w : PMIOPort  Port=5  Side=Right
  wires:
  gate_commands/1 -> Simulink-PS Converter/1
  connections:
  Three-Phase Bridge (ideal)/LConn1 -- udc(+)/RConn1
  Three-Phase Bridge (ideal)/RConn3 -- w/RConn1
  Three-Phase Bridge (ideal)/RConn2 -- v/RConn1
  Three-Phase Bridge (ideal)/LConn2 -- udc(-)/RConn1
  Three-Phase Bridge (ideal)/RConn1 -- u/RConn1
  Simulink-PS Converter/RConn1 -- Three-Phase Bridge (ideal)/RConn4
  PS Terminator/LConn1 -- Three-Phase Bridge (ideal)/LConn3
  PS Terminator1/LConn1 -- Three-Phase Bridge (ideal)/LConn4

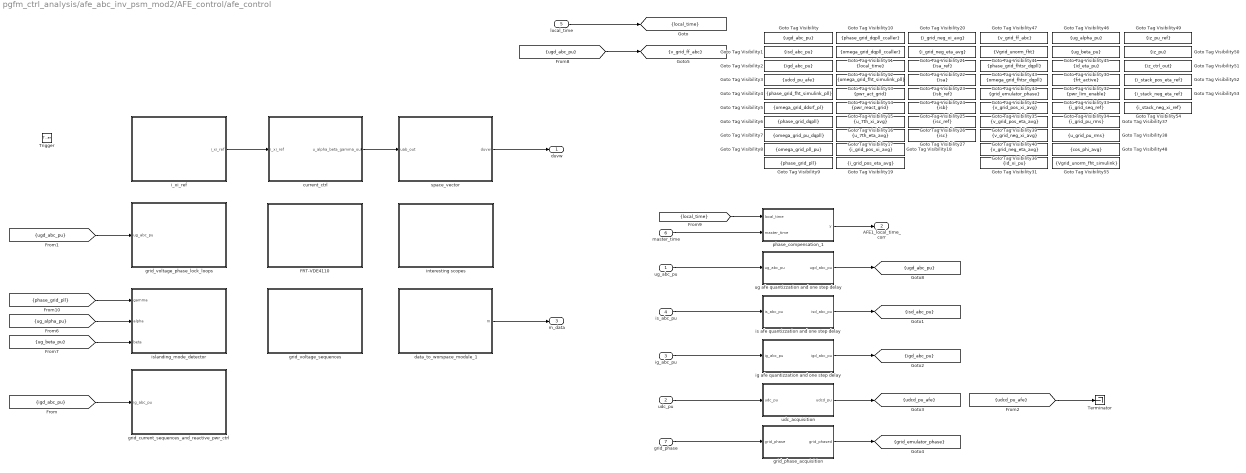
== system pgfm_ctrl_analysis/afe_abc_inv_psm_mod2/AFE_control/afe_control ==
  ug_abc_pu : Inport
  udc_pu : Inport  Port=2
  ig_abc_pu : Inport  Port=3
  is_abc_pu : Inport  Port=4
  local_time : Inport  Port=5
  master_time : Inport  Port=6
  grid_phase : Inport  Port=7
  Trigger : TriggerPort  VariantControl=(inherit)  PortDimensions=1
  FRT-VDE4110 : Subsystem
  Goto Tag Visibility : GotoTagVisibility  GotoTag=ugd_abc_pu
  Goto Tag Visibility1 : GotoTagVisibility  GotoTag=isd_abc_pu
  Goto Tag Visibility10 : GotoTagVisibility  GotoTag=phase_grid_dqpll_ccaller
  Goto Tag Visibility11 : GotoTagVisibility  GotoTag=omega_grid_dqpll_ccaller
  Goto Tag Visibility12 : GotoTagVisibility  GotoTag=local_time
  Goto Tag Visibility13 : GotoTagVisibility  GotoTag=omega_grid_fht_simulink_pll
  Goto Tag Visibility14 : GotoTagVisibility  GotoTag=pwr_act_grid
  Goto Tag Visibility15 : GotoTagVisibility  GotoTag=pwr_react_grid
  Goto Tag Visibility16 : GotoTagVisibility  GotoTag=u_7th_xi_avg
  Goto Tag Visibility17 : GotoTagVisibility  GotoTag=u_7th_eta_avg
  Goto Tag Visibility18 : GotoTagVisibility  GotoTag=i_grid_pos_xi_avg
  Goto Tag Visibility19 : GotoTagVisibility  GotoTag=i_grid_pos_eta_avg
  Goto Tag Visibility2 : GotoTagVisibility  GotoTag=igd_abc_pu
  Goto Tag Visibility20 : GotoTagVisibility  GotoTag=i_grid_neg_xi_avg
  Goto Tag Visibility21 : GotoTagVisibility  GotoTag=i_grid_neg_eta_avg
  Goto Tag Visibility22 : GotoTagVisibility  GotoTag=isa_ref
  Goto Tag Visibility23 : GotoTagVisibility  GotoTag=isa
  Goto Tag Visibility24 : GotoTagVisibility  GotoTag=isb_ref
  Goto Tag Visibility25 : GotoTagVisibility  GotoTag=isb
  Goto Tag Visibility26 : GotoTagVisibility  GotoTag=isc_ref
  Goto Tag Visibility27 : GotoTagVisibility  GotoTag=isc
  Goto Tag Visibility3 : GotoTagVisibility  GotoTag=udcd_pu_afe
  Goto Tag Visibility30 : GotoTagVisibility  GotoTag=id_eta_pu
  Goto Tag Visibility31 : GotoTagVisibility  GotoTag=id_xi_pu
  Goto Tag Visibility32 : GotoTagVisibility  GotoTag=frt_active
  Goto Tag Visibility33 : GotoTagVisibility  GotoTag=pwr_lim_enable
  Goto Tag Visibility34 : GotoTagVisibility  GotoTag=i_grid_seq_ref
  Goto Tag Visibility35 : GotoTagVisibility  GotoTag=v_grid_pos_xi_avg
  Goto Tag Visibility36 : GotoTagVisibility  GotoTag=v_grid_neg_eta_avg
  Goto Tag Visibility37 : GotoTagVisibility  GotoTag=i_grid_pu_rms
  Goto Tag Visibility38 : GotoTagVisibility  GotoTag=u_grid_pu_rms
  Goto Tag Visibility39 : GotoTagVisibility  GotoTag=v_grid_pos_eta_avg
  Goto Tag Visibility4 : GotoTagVisibility  GotoTag=phase_grid_fht_simulink_pll
  Goto Tag Visibility40 : GotoTagVisibility  GotoTag=v_grid_neg_xi_avg
  Goto Tag Visibility41 : GotoTagVisibility  GotoTag=Vgrid_unorm_fht
  Goto Tag Visibility42 : GotoTagVisibility  GotoTag=grid_emulator_phase
  Goto Tag Visibility43 : GotoTagVisibility  GotoTag=phase_grid_fhtsr_dqpll
  Goto Tag Visibility44 : GotoTagVisibility  GotoTag=omega_grid_fhtsr_dqpll
  Goto Tag Visibility45 : GotoTagVisibility  GotoTag=ug_beta_pu
  Goto Tag Visibility46 : GotoTagVisibility  GotoTag=ug_alpha_pu
  Goto Tag Visibility47 : GotoTagVisibility  GotoTag=v_grid_ff_abc
  Goto Tag Visibility48 : GotoTagVisibility  GotoTag=cos_phi_avg
  Goto Tag Visibility49 : GotoTagVisibility  GotoTag=iz_pu_ref
  Goto Tag Visibility5 : GotoTagVisibility  GotoTag=omega_grid_ddsrf_pl
  Goto Tag Visibility50 : GotoTagVisibility  GotoTag=iz_pu
  Goto Tag Visibility51 : GotoTagVisibility  GotoTag=iz_ctrl_out
  Goto Tag Visibility52 : GotoTagVisibility  GotoTag=i_stack_pos_eta_ref
  Goto Tag Visibility53 : GotoTagVisibility  GotoTag=i_stack_neg_eta_ref
  Goto Tag Visibility54 : GotoTagVisibility  GotoTag=i_stack_neg_xi_ref
  Goto Tag Visibility55 : GotoTagVisibility  GotoTag=Vgrid_unorm_fht_simulink
  Goto Tag Visibility6 : GotoTagVisibility  GotoTag=phase_grid_dqpll
  Goto Tag Visibility7 : GotoTagVisibility  GotoTag=omega_grid_pu_dqpll
  Goto Tag Visibility8 : GotoTagVisibility  GotoTag=omega_grid_pll_pu
  Goto Tag Visibility9 : GotoTagVisibility  GotoTag=phase_grid_pll
  Terminator : Terminator
  current_ctrl : Subsystem
  data_to_worspace_module_1 : Subsystem
  grid_current_sequences_and_reactive_pwr_ctrl : Subsystem
  grid_phase_acquisition : Subsystem
  grid_voltage_phase_lock_loops : Subsystem
  grid_voltage_sequences : Subsystem
  i_xi_ref : Subsystem
  ig afe quantizzation and one step delay : Subsystem
  interesting scopes : Subsystem
  is afe quantizzation and one step delay : Subsystem
  islanding_mode_detector : Subsystem
  phase_compensation_1 : Subsystem
  space_vector : Subsystem
  udc_acquisition : Subsystem
  ug afe quantizzation and one step delay : Subsystem
  duvw : Outport
  AFE1_local_time_corr : Outport  Port=2
  m_data : Outport  Port=3
  tag scope: grid_emulator_phase=scoped, igd_abc_pu=scoped, isd_abc_pu=scoped, local_time=scoped, udcd_pu_afe=scoped, ugd_abc_pu=scoped, v_grid_ff_abc=scoped
  wires:
  i_xi_ref/1(i_xi_ref) -> current_ctrl/1(i_xi_ref)
  current_ctrl/1(u_alpha_beta_gamma_out) -> space_vector/1(uab_out)
  [udcd_pu_afe] -> Terminator/1
  data_to_worspace_module_1/1(m) -> m_data/1
  [ugd_abc_pu] -> [v_grid_ff_abc]
  grid_phase_acquisition/1(grid_phased) -> [grid_emulator_phase]
  grid_phase/1 -> grid_phase_acquisition/1(grid_phase)
  [local_time] -> phase_compensation_1/1(local_time)
  phase_compensation_1/1(y) -> AFE1_local_time_corr/1
  master_time/1 -> phase_compensation_1/2(master_time)
  local_time/1 -> [local_time]
  [ug_beta_pu] -> islanding_mode_detector/3(beta)
  ig afe quantizzation and one step delay/1(igd_abc_pu) -> [igd_abc_pu]
  is afe quantizzation and one step delay/1(isd_abc_pu) -> [isd_abc_pu]
  ug afe quantizzation and one step delay/1(ugd_abc_pu) -> [ugd_abc_pu]
  [ug_alpha_pu] -> islanding_mode_detector/2(alpha)
  [phase_grid_pll] -> islanding_mode_detector/1(gamma)
  udc_acquisition/1(udcd_pu) -> [udcd_pu_afe]
  udc_pu/1 -> udc_acquisition/1(udc_pu)
  [igd_abc_pu] -> grid_current_sequences_and_reactive_pwr_ctrl/1(ig_abc_pu)
  [ugd_abc_pu] -> grid_voltage_phase_lock_loops/1(ug_abc_pu)
  ig_abc_pu/1 -> ig afe quantizzation and one step delay/1(ig_abc_pu)
  is_abc_pu/1 -> is afe quantizzation and one step delay/1(is_abc_pu)
  space_vector/1(duvw) -> duvw/1
  ug_abc_pu/1 -> ug afe quantizzation and one step delay/1(ug_abc_pu)

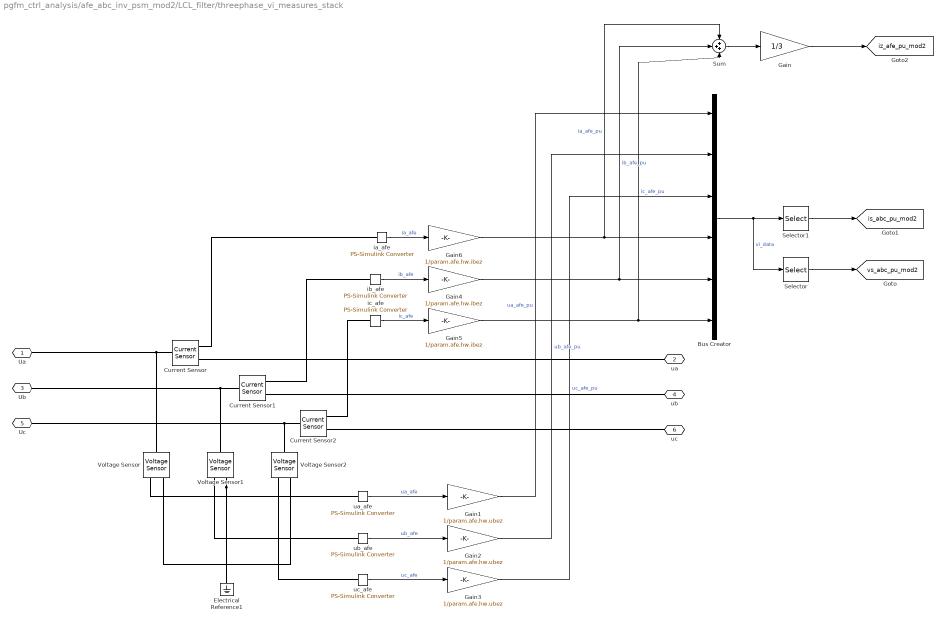
== system pgfm_ctrl_analysis/afe_abc_inv_psm_mod2/LCL_filter/threephase_vi_measures_stack ==
  Bus Creator : BusCreator  Inputs=6
  Current Sensor : fl_lib/Electrical/Electrical Sensors/Current Sensor
  Current Sensor1 : fl_lib/Electrical/Electrical Sensors/Current Sensor
  Current Sensor2 : fl_lib/Electrical/Electrical Sensors/Current Sensor
  Electrical Reference1 : fl_lib/Electrical/Electrical Elements/Electrical Reference
  Gain : Gain  Gain=1/3
  Gain1 : Gain  Gain=1/param.afe.hw.ubez
  Gain2 : Gain  Gain=1/param.afe.hw.ubez
  Gain3 : Gain  Gain=1/param.afe.hw.ubez
  Gain4 : Gain  Gain=1/param.afe.hw.ibez
  Gain5 : Gain  Gain=1/param.afe.hw.ibez
  Gain6 : Gain  Gain=1/param.afe.hw.ibez
  Selector : Selector  InputPortWidth=6  IndexOptions=Index vector (dialog)  Indices=[1 2 3]  OutputSizes=1  RuntimeRangeChecks=off
  Selector1 : Selector  InputPortWidth=6  IndexOptions=Index vector (dialog)  Indices=[4 5 6]  OutputSizes=1  RuntimeRangeChecks=off
  Sum : Sum  Inputs=+++
  Voltage Sensor : fl_lib/Electrical/Electrical Sensors/Voltage Sensor
  Voltage Sensor1 : fl_lib/Electrical/Electrical Sensors/Voltage Sensor
  Voltage Sensor2 : fl_lib/Electrical/Electrical Sensors/Voltage Sensor
  ia_afe : nesl_utility/PS-Simulink Converter  PhysicalDomain=network_engine_domain  SubClassName=ps_output  LeftPortType=input  RightPortType=output  PseudoPeriodic=off  Frequencies=[]  VectorFormat=1-D array  Unit=A  AffineConversion=off
  ib_afe : nesl_utility/PS-Simulink Converter  PhysicalDomain=network_engine_domain  SubClassName=ps_output  LeftPortType=input  RightPortType=output  PseudoPeriodic=off  Frequencies=[]  VectorFormat=1-D array  Unit=A  AffineConversion=off
  ic_afe : nesl_utility/PS-Simulink Converter  PhysicalDomain=network_engine_domain  SubClassName=ps_output  LeftPortType=input  RightPortType=output  PseudoPeriodic=off  Frequencies=[]  VectorFormat=1-D array  Unit=A  AffineConversion=off
  ua_afe : nesl_utility/PS-Simulink Converter  PhysicalDomain=network_engine_domain  SubClassName=ps_output  LeftPortType=input  RightPortType=output  PseudoPeriodic=off  Frequencies=[]  VectorFormat=1-D array  Unit=V  AffineConversion=off
  ub_afe : nesl_utility/PS-Simulink Converter  PhysicalDomain=network_engine_domain  SubClassName=ps_output  LeftPortType=input  RightPortType=output  PseudoPeriodic=off  Frequencies=[]  VectorFormat=1-D array  Unit=V  AffineConversion=off
  uc_afe : nesl_utility/PS-Simulink Converter  PhysicalDomain=network_engine_domain  SubClassName=ps_output  LeftPortType=input  RightPortType=output  PseudoPeriodic=off  Frequencies=[]  VectorFormat=1-D array  Unit=V  AffineConversion=off
  Ua : PMIOPort  Side=Left
  ua : PMIOPort  Port=2  Side=Right
  Ub : PMIOPort  Port=3  Side=Left
  ub : PMIOPort  Port=4  Side=Right
  Uc : PMIOPort  Port=5  Side=Left
  uc : PMIOPort  Port=6  Side=Right
  tag scope: is_abc_pu_mod2=global, iz_afe_pu_mod2=global, vs_abc_pu_mod2=global
  wires:
  Gain5/1 -> Sum/3, Bus Creator/6  "ic_afe_pu"
  Gain4/1 -> Bus Creator/5, Sum/2  "ib_afe_pu"
  Gain6/1 -> Bus Creator/4, Sum/1  "ia_afe_pu"
  Gain3/1 -> Bus Creator/3  "uc_afe_pu"
  Gain2/1 -> Bus Creator/2  "ub_afe_pu"
  Gain1/1 -> Bus Creator/1  "ua_afe_pu"
  Gain/1 -> [iz_afe_pu_mod2]
  Sum/1 -> Gain/1
  Selector1/1 -> [is_abc_pu_mod2]
  uc_afe/1 -> Gain3/1  "uc_afe"
  ub_afe/1 -> Gain2/1  "ub_afe"
  ua_afe/1 -> Gain1/1  "ua_afe"
  ic_afe/1 -> Gain5/1  "ic_afe"
  ia_afe/1 -> Gain6/1  "ia_afe"
  ib_afe/1 -> Gain4/1  "ib_afe"
  Selector/1 -> [vs_abc_pu_mod2]
  Bus Creator/1 -> Selector1/1, Selector/1  "vi_data"
  connections:
  Current Sensor2/RConn2 -- uc/RConn1
  ic_afe/LConn1 -- Current Sensor2/RConn1
  ia_afe/LConn1 -- Current Sensor/RConn1
  ib_afe/LConn1 -- Current Sensor1/RConn1
  Voltage Sensor2/RConn1 -- uc_afe/LConn1
  Current Sensor1/RConn2 -- ub/RConn1
  Voltage Sensor/LConn1 -- Ua/RConn1 -- Current Sensor/LConn1
  Current Sensor2/LConn1 -- Uc/RConn1 -- Voltage Sensor2/LConn1
  Voltage Sensor1/RConn1 -- ub_afe/LConn1
  Current Sensor/RConn2 -- ua/RConn1
  Voltage Sensor/RConn1 -- ua_afe/LConn1
  Voltage Sensor1/RConn2 -- Voltage Sensor2/RConn2 -- Voltage Sensor/RConn2 -- Electrical Reference1/LConn1
  Voltage Sensor1/LConn1 -- Ub/RConn1 -- Current Sensor1/LConn1

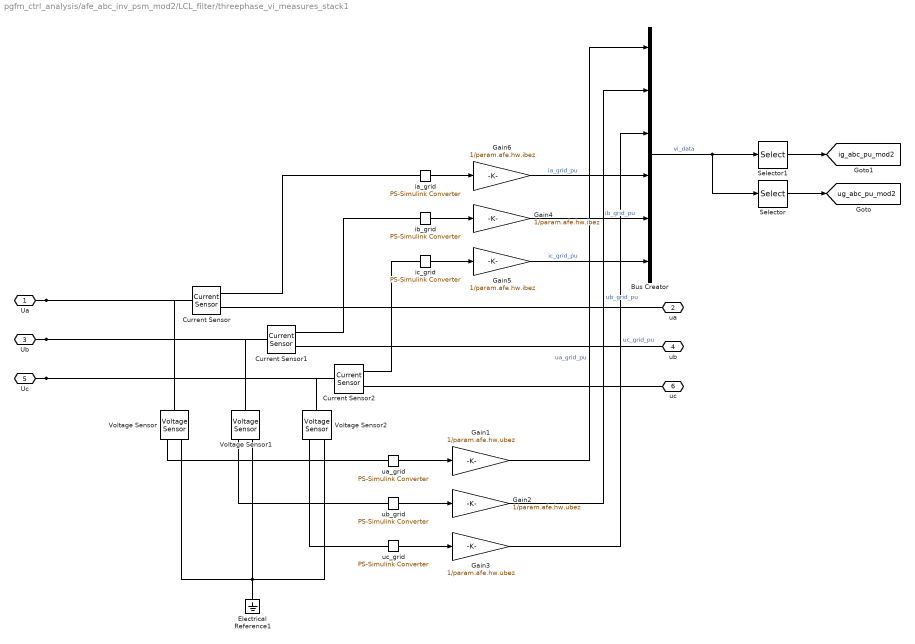
== system pgfm_ctrl_analysis/afe_abc_inv_psm_mod2/LCL_filter/threephase_vi_measures_stack1 ==
  Bus Creator : BusCreator  Inputs=6
  Current Sensor : fl_lib/Electrical/Electrical Sensors/Current Sensor
  Current Sensor1 : fl_lib/Electrical/Electrical Sensors/Current Sensor
  Current Sensor2 : fl_lib/Electrical/Electrical Sensors/Current Sensor
  Electrical Reference1 : fl_lib/Electrical/Electrical Elements/Electrical Reference
  Gain1 : Gain  Gain=1/param.afe.hw.ubez
  Gain2 : Gain  Gain=1/param.afe.hw.ubez
  Gain3 : Gain  Gain=1/param.afe.hw.ubez
  Gain4 : Gain  Gain=1/param.afe.hw.ibez
  Gain5 : Gain  Gain=1/param.afe.hw.ibez
  Gain6 : Gain  Gain=1/param.afe.hw.ibez
  Selector : Selector  InputPortWidth=6  IndexOptions=Index vector (dialog)  Indices=[1 2 3]  OutputSizes=1  RuntimeRangeChecks=off
  Selector1 : Selector  InputPortWidth=6  IndexOptions=Index vector (dialog)  Indices=[4 5 6]  OutputSizes=1  RuntimeRangeChecks=off
  Voltage Sensor : fl_lib/Electrical/Electrical Sensors/Voltage Sensor
  Voltage Sensor1 : fl_lib/Electrical/Electrical Sensors/Voltage Sensor
  Voltage Sensor2 : fl_lib/Electrical/Electrical Sensors/Voltage Sensor
  ia_grid : nesl_utility/PS-Simulink Converter  PhysicalDomain=network_engine_domain  SubClassName=ps_output  LeftPortType=input  RightPortType=output  PseudoPeriodic=off  Frequencies=[]  VectorFormat=1-D array  Unit=A  AffineConversion=off
  ib_grid : nesl_utility/PS-Simulink Converter  PhysicalDomain=network_engine_domain  SubClassName=ps_output  LeftPortType=input  RightPortType=output  PseudoPeriodic=off  Frequencies=[]  VectorFormat=1-D array  Unit=A  AffineConversion=off
  ic_grid : nesl_utility/PS-Simulink Converter  PhysicalDomain=network_engine_domain  SubClassName=ps_output  LeftPortType=input  RightPortType=output  PseudoPeriodic=off  Frequencies=[]  VectorFormat=1-D array  Unit=A  AffineConversion=off
  ua_grid : nesl_utility/PS-Simulink Converter  PhysicalDomain=network_engine_domain  SubClassName=ps_output  LeftPortType=input  RightPortType=output  PseudoPeriodic=off  Frequencies=[]  VectorFormat=1-D array  Unit=V  AffineConversion=off
  ub_grid : nesl_utility/PS-Simulink Converter  PhysicalDomain=network_engine_domain  SubClassName=ps_output  LeftPortType=input  RightPortType=output  PseudoPeriodic=off  Frequencies=[]  VectorFormat=1-D array  Unit=V  AffineConversion=off
  uc_grid : nesl_utility/PS-Simulink Converter  PhysicalDomain=network_engine_domain  SubClassName=ps_output  LeftPortType=input  RightPortType=output  PseudoPeriodic=off  Frequencies=[]  VectorFormat=1-D array  Unit=V  AffineConversion=off
  Ua : PMIOPort  Side=Left
  ua : PMIOPort  Port=2  Side=Right
  Ub : PMIOPort  Port=3  Side=Left
  ub : PMIOPort  Port=4  Side=Right
  Uc : PMIOPort  Port=5  Side=Left
  uc : PMIOPort  Port=6  Side=Right
  tag scope: ig_abc_pu_mod2=global, ug_abc_pu_mod2=global
  wires:
  Gain5/1 -> Bus Creator/6  "ic_grid_pu"
  Gain4/1 -> Bus Creator/5  "ib_grid_pu"
  Gain6/1 -> Bus Creator/4  "ia_grid_pu"
  Gain3/1 -> Bus Creator/3  "uc_grid_pu"
  Gain2/1 -> Bus Creator/2  "ub_grid_pu"
  Gain1/1 -> Bus Creator/1  "ua_grid_pu"
  Bus Creator/1 -> Selector/1, Selector1/1  "vi_data"
  Selector/1 -> [ug_abc_pu_mod2]
  ib_grid/1 -> Gain4/1
  ia_grid/1 -> Gain6/1
  ic_grid/1 -> Gain5/1
  ua_grid/1 -> Gain1/1
  ub_grid/1 -> Gain2/1
  uc_grid/1 -> Gain3/1
  Selector1/1 -> [ig_abc_pu_mod2]
  connections:
  Ub/RConn1 -- Current Sensor1/LConn1 -- Voltage Sensor1/LConn1
  Electrical Reference1/LConn1 -- Voltage Sensor/RConn2 -- Voltage Sensor2/RConn2 -- Voltage Sensor1/RConn2
  Voltage Sensor/RConn1 -- ua_grid/LConn1
  Current Sensor/RConn2 -- ua/RConn1
  Voltage Sensor1/RConn1 -- ub_grid/LConn1
  Uc/RConn1 -- Voltage Sensor2/LConn1 -- Current Sensor2/LConn1
  Ua/RConn1 -- Current Sensor/LConn1 -- Voltage Sensor/LConn1
  Current Sensor1/RConn2 -- ub/RConn1
  Voltage Sensor2/RConn1 -- uc_grid/LConn1
  ib_grid/LConn1 -- Current Sensor1/RConn1
  ia_grid/LConn1 -- Current Sensor/RConn1
  ic_grid/LConn1 -- Current Sensor2/RConn1
  Current Sensor2/RConn2 -- uc/RConn1

== system pgfm_ctrl_analysis/afe_abc_inv_psm_mod2/afe/sv_pwm ==
  duties_uvw : Inport
  Bus Selector2 : BusSelector  OutputSignals=du(k),dv(k),dw(k)
  Constant1 : Constant  Value=param.afe.behav.pwm_phase_shift_mod2
  modulator1 : Subsystem
  td2tc_1 : TransferFcn  Denominator=[param.glb_time.tc 1]
  td2tc_2 : TransferFcn  Denominator=[param.glb_time.tc 1]
  td2tc_3 : TransferFcn  Denominator=[param.glb_time.tc 1]
  gate_cmds : Outport
  wires:
  td2tc_2/1 -> modulator1/2(v)  "dv(t)"
  td2tc_3/1 -> modulator1/3(w)  "dw(t)"
  td2tc_1/1 -> modulator1/1(u)  "du(t)"
  duties_uvw/1 -> Bus Selector2/1
  Bus Selector2/3 -> td2tc_3/1  "<dw(k)>"
  Bus Selector2/2 -> td2tc_2/1  "<dv(k)>"
  Bus Selector2/1 -> td2tc_1/1  "<du(k)>"
  Constant1/1 -> modulator1/4(phase)
  modulator1/1(gate_cmds) -> gate_cmds/1
